simulink model "underactuated_manipulator"  (R2025b)
settings: Solver=VariableStepAuto  StartTime=0.0  StopTime=20.0  RelTol=1e-3
settings Model: Creator=Vishrut  LastModifiedBy=Vishrut

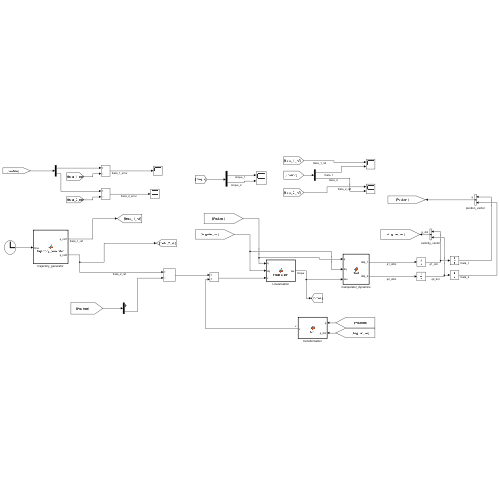
[thumbnail: Simulink's stored preview of the top-level diagram]
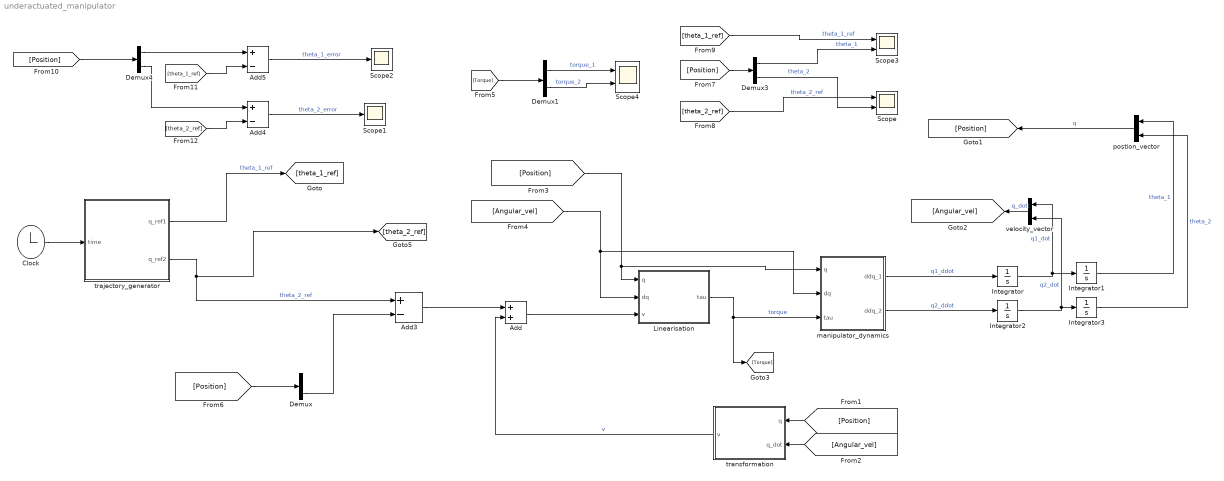
== system underactuated_manipulator ==
  Add : Sum
  Add3 : Sum  Inputs=+-
  Add4 : Sum  Inputs=+-
  Add5 : Sum  Inputs=+-
  Clock : Clock
  Demux{,1,3..4} (4 alike) : Demux  Outputs=2
  Integrator : Integrator
  Integrator1 : Integrator  InitialCondition=1.0
  Integrator2 : Integrator
  Integrator3 : Integrator  InitialCondition=0.5708
  Linearisation : MATLAB Function  TreatAsAtomicUnit=on
  Scope : Scope  NumInputPorts=2
      settings: ActiveDisplayYMinimum=0.57074967443740909  ActiveDisplayYMaximum=0.57080559172917678
  Scope1 : Scope
      settings: ActiveDisplayYMinimum=-1  ActiveDisplayYMaximum=1
  Scope2 : Scope
      settings: ActiveDisplayYMinimum=-0.48508163662911419  ActiveDisplayYMaximum=1.4822543646177151  DataLoggingVariableName=ScopeData2
  Scope3 : Scope  NumInputPorts=2
      settings: ActiveDisplayYMinimum=0.99999512503314625  ActiveDisplayYMaximum=1.0000438747016835  DataLoggingVariableName=ScopeData3
  Scope4 : Scope  NumInputPorts=2
      settings: ActiveDisplayYMinimum=-3.2148733434426431  ActiveDisplayYMaximum=28.933860090983796  DataLoggingVariableName=ScopeData4
  manipulator_dynamics : MATLAB Function  TreatAsAtomicUnit=on
  postion_vector : Concatenate
  trajectory_generator : MATLAB Function  TreatAsAtomicUnit=on
  transformation : MATLAB Function  TreatAsAtomicUnit=on
  velocity_vector : Concatenate
  wires:
  [Position] -> transformation/1(q)
  Add5/1 -> Scope2/1  "theta_1_error"
  Demux4/2 -> Add4/1
  [theta_2_ref] -> Add4/2
  [Angular_vel] -> Linearisation/2(dq), manipulator_dynamics/2(dq)
  Integrator1/1 -> postion_vector/1  "theta_1"
  manipulator_dynamics/1(ddq_1) -> Integrator/1  "q1_ddot"
  Integrator/1 -> velocity_vector/1, Integrator1/1  "q1_dot"
  Demux4/1 -> Add5/1
  [Angular_vel] -> transformation/2(q_dot)
  Add4/1 -> Scope1/1  "theta_2_error"
  velocity_vector/1 -> [Angular_vel]  "q_dot"
  manipulator_dynamics/2(ddq_2) -> Integrator2/1  "q2_ddot"
  postion_vector/1 -> [Position]  "q"
  Clock/1 -> trajectory_generator/1(time)
  [Position] -> Linearisation/1(q), manipulator_dynamics/1(q)
  Linearisation/1(tau) -> [Torque], manipulator_dynamics/3(tau)  "torque"
  [Position] -> Demux4/1
  Integrator2/1 -> velocity_vector/2, Integrator3/1  "q2_dot"
  [theta_1_ref] -> Add5/2
  [Position] -> Demux3/1
  trajectory_generator/2(q_ref2) -> Add3/1, [theta_2_ref]  "theta_2_ref"
  [theta_1_ref] -> Scope3/1  "theta_1_ref"
  Add3/1 -> Add/1
  Demux3/1 -> Scope3/2  "theta_1"
  Integrator3/1 -> postion_vector/2  "theta_2"
  Add/1 -> Linearisation/3(v)
  [Torque] -> Demux1/1
  Demux/2 -> Add3/2
  trajectory_generator/1(q_ref1) -> [theta_1_ref]  "theta_1_ref"
  Demux1/1 -> Scope4/1  "torque_1"
  Demux1/2 -> Scope4/2  "torque_2"
  [Position] -> Demux/1
  transformation/1(v) -> Add/2  "v"
  Demux3/2 -> Scope/2  "theta_2"
  [theta_2_ref] -> Scope/1  "theta_2_ref"

== matlab function underactuated_manipulator/Linearisation ==
  data: q input size=[2 1]; dq input size=[2 1]; v input; tau output size=[2 1]
function tau = linearisation(q, dq, v)
   
    r1 = 1.0; r2 = 0.8;         
    m1 = 0.5; m2 = 1.5;         
    J1 = 5.0; J2 = 5.0;         
    g  = 9.8;                   
    
    q1 = q(1); q2 = q(2);
    dq1 = dq(1); dq2 = dq(2);
    m11 = J1 + J2 + m1*r1^2 + m2*(r1^2 + r2^2 + 2*r1*r2*cos(q2));
    m12 = J2 + m2*(r2^2 + r1*r2*cos(q2));
    m21 = m12;
    m22 = J2 + m2*r2^2;
    h = m2*r1*r2*sin(q2);
    c1 = -h*(2*dq1*dq2 + dq2^2);
    c2 = h*dq1^2;
    g1 = (m1+m2)*g*r1*cos(q1) + m2*g*r2*cos(q1+q2);
    g2 = m2*g*r2*cos(q1+q2);
    gain_alpha = (m12 - (m11*m22)/m21);
    drift_beta = (c1 + g1) - (m11/m21)*(c2 + g2);
    tau1 = gain_alpha * v + drift_beta;
    tau = [tau1;0];
end

== matlab function underactuated_manipulator/manipulator_dynamics ==
  data: q input size=[2 1]; dq input size=[2 1]; tau input size=[2 1]; ddq_1 output; ddq_2 output
function [ddq_1,ddq_2] = plant(q, dq, tau)
   
    r1 = 1.0; r2 = 0.8;         
    m1 = 0.5; m2 = 1.5;         
    J1 = 5.0; J2 = 5.0;         
    g  = 9.8;                   
    
   
    q1 = q(1); q2 = q(2);
    dq1 = dq(1); dq2 = dq(2);
    m11 = J1 + J2 + m1*r1^2 + m2*(r1^2 + r2^2 + 2*r1*r2*cos(q2));
    m12 = J2 + m2*(r2^2 + r1*r2*cos(q2));
    m21 = m12;
    m22 = J2 + m2*r2^2;
    M = [m11, m12; m21, m22];
    h = m2*r1*r2*sin(q2);
    C_vec = [-h*(2*dq1*dq2 + dq2^2); 
              h*dq1^2];
    g1 = (m1+m2)*g*r1*cos(q1) + m2*g*r2*cos(q1+q2);
    g2 = m2*g*r2*cos(q1+q2);
    G_vec = [g1; g2];
    Total_Torque = tau;
    ddq = M \ (Total_Torque - C_vec - G_vec);
    ddq_1 = ddq(1);
    ddq_2 = ddq(2);

end

== matlab function underactuated_manipulator/trajectory_generator ==
  data: time input; q_ref1 output; q_ref2 output
function [q_ref1,q_ref2] = trajectory_generator(time)


q_ref1 = 1.0;

q_ref2 = 0.5708;





end

== matlab function underactuated_manipulator/transformation ==
  data: q input size=[2 1]; v output; q_dot input size=[2 1]
function v = fcn(q, q_dot)

 q1e = 1.0;
  q2e = pi/2 - 1.0;
    
    x = [q(1); q(2); q_dot(1); q_dot(2)];
    x_eq = [q1e; q2e; 0; 0];
    K = [268.4489  257.9608  206.6531  184.9319];
    v = -K * (x - x_eq);

end
